simulink model "ball_balancing_omni3_multibody_lqi_rev1_r2024b"  (R2024b)
settings: Solver=VariableStepAuto  StartTime=0.0  StopTime=50  MaxStep=1e-3  MinStep=1e-6  RelTol=ballbotParams.simulation.relativeTolerance
PreLoadFcn:
  | if ~exist('ballbotParams','var'), ballbotParams = ballbotRev1Parameters; end
InitFcn:
  | if ~exist('ballbotParams','var') || ~isfield(ballbotParams,'parameterSource') || ballbotParams.parameterSource ~= "ballbotRev1Parameters" || ~isfield(ballbotParams,'controller') || ~isfield(ballbotParams,'estimator') || ~isfield(ballbotParams.controller,'torqueDrive') || ~isfield(ballbotParams.controller.torqueDrive,'propulsionGain') || ~isfield(ballbotParams.estimator,'truthDelaySteps') || ~isfield(ballbotParams.controller.torqueLqi,'robustness'), ballbotParams = ballbotRev1Parameters; end
  | % ballbotRev1RuntimeApply: re-apply runtime solver/driver/plant settings on every sim start.
  | clear functions;
  | ballbotRev1SimConfig;
  | if exist('ballbotParams','var'), ballbotRev1PlantAugment(bdroot, ballbotParams); end
values from neighbouring files (symbols this model uses):
  N = 0    [ballbotRollingResistance.m]
  s = result.spec    [ballbotBenchmark.m]
undefined symbols (not defined in the file or in its folder): ballbotCustomFriction, ballbotEstimatorInitialState, ballbotEstimatorUpdate, ballbotEulerToQuaternion, ballbotImuFromJoint, ballbotLqiControllerUpdate, ballbotLqiFeedbackState, ballbotMdd3aGateDrive, ballbotParams, ballbotPoseFromJoint, ballbotRev1CommandProfile, ballbotRollingResistance, ballbotRoverInitialPosition, ballbotShaftFrictionTorque, ballbotTorqueDutyStep, ballbotTruthGate, ballbotWheelRateFromDisplacement, X, Y, Z
libraries: nesl_utility x54, sm_lib x28, fl_lib x21, ee_lib x6
(part 1 of 3)
settings Model: Creator=cafdr  LastModifiedBy=cafdr
settings DataIOCC: LoggingIntervals=[-inf,inf]
settings ModelReferenceCC: UpdateModelReferenceTargets=IfOutOfDate
settings ConfigComp: CovBoundaryAbsTol=1.0e-5
settings SimscapeCC: SimscapeNominalValues="[{\"value\":\"1\",\"unit\":\"A\"},{\"value\":\"1\",\"unit\":\"bar\"},{\"value\":\"1\",\"unit\":\"cm^2\"},{\"value\":\"1\",\"unit\":\"cm^3/s\"},{\"value\":\"1\",\"unit\":\"kJ/kg\"},{\"value\":\"1\",\"unit\":\"kW\"},{\"value\":\"1\",\"unit\":\"l\"},{\"value\":\"1\",\"unit\":\"N\"},{\"value\":\"1\",\"unit\":\"N*m\"},{\"value\":\"1\",\"unit\":\"V\"},{\"value\":\"0.001\",\"unit\":\"Wb\"}]"  SimscapeLogDataHistory=10000
settings ExplorerConfigSet: InternalSimMechanicsExplorerSettings=|
  | <ExplorerConfiguration>
  | 
  |   <canonicalview>default</canonicalview>
  | 
  |   <TilePanel>
  |     <TileInfo>
  |       <Tiles Columns="1" Count="1" Height="986" Rows="1" Width="1142">
  |         <Row Weight="1"/>
  |         <Column Weight="1"/>
  |         <Tile Height="1" Width="1" X="0" Y="0"/>
  |       </Tiles>
  |     </TileInfo>
  |     <SceneInfo>
  |       <SceneViewer>
  |         <IsThisViewStd>
  |           <IsStandardView>off</IsStandardView>
  |           <StandardViewName>Front</StandardViewName>
  |         </IsThisViewStd>
  |         <BGColor>
  |           <R>1</R>
  |           <G>1</G>
  |           <B>1</B>
  |           <A>1</A>
  |         </BGColor>
  |         <Camera>
  |           <DoPerspective>off</DoPerspective>
  |           <Position>
  |             <X>1.5473752302641908</X>
  |             <Y>-7.8906176009490112</Y>
  |             <Z>3.2187132461389409</Z>
  |           </Position>
  |           <Center>
  |             <X>-0.24631476973580918</X>
  |             <Y>-0.11269760094901093</Y>
  |             <Z>0.28416324613894073</Z>
  |           </Center>
  |           <Up>
  |             <X>-0.21384970147003254</X>
  |             <Y>0.30128090391364881</Y>
  |             <Z>0.92924599655750617</Z>
  |           </Up>
  |           <XLim>0.70155682369920191</XLim>
  |           <YLim>0.70155682369920191</YLim>
  |           <ViewLimDist>0.01</ViewLimDist>
  |         </Camera>
  |       </SceneViewer>
  |     </SceneInfo>
  |   </TilePanel>
  | 
  |   <MechEditorPanel>
  |     <GfxPanelCameraMap/>
  |     <Cameras/>
  |     <VideoCreator>
  |       <IncludeTiles>All</IncludeTiles>
  |       <IncludeTime>on</IncludeTime>
  |       <IncludeWorldFrame>off</IncludeWorldFrame>
  |       <PlaybackSpeedRatio>1</PlaybackSpeedRatio>
  |       <FrameRate>30</FrameRate>
  |       <FrameSize>auto</FrameSize>
  |       <VideoFormat>UncompressedAVI</VideoFormat>
  |     </VideoCreator>
  |   </MechEditorPanel>
  | 
  |   <PlaybackSettings>
  |     <PlaybackSpeedFactor>1</PlaybackSpeedFactor>
  |   </PlaybackSettings>
  | 
  | </ExplorerConfiguration>

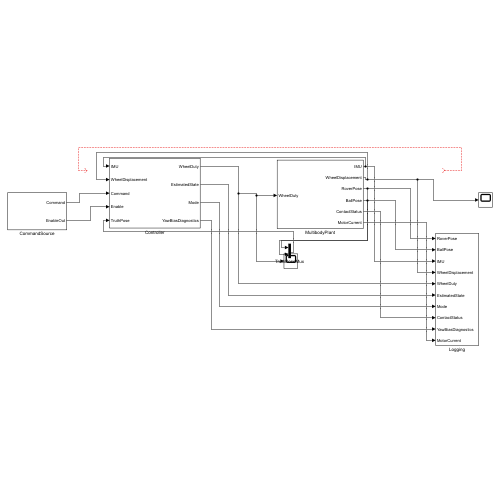
[thumbnail: Simulink's stored preview of the top-level diagram]
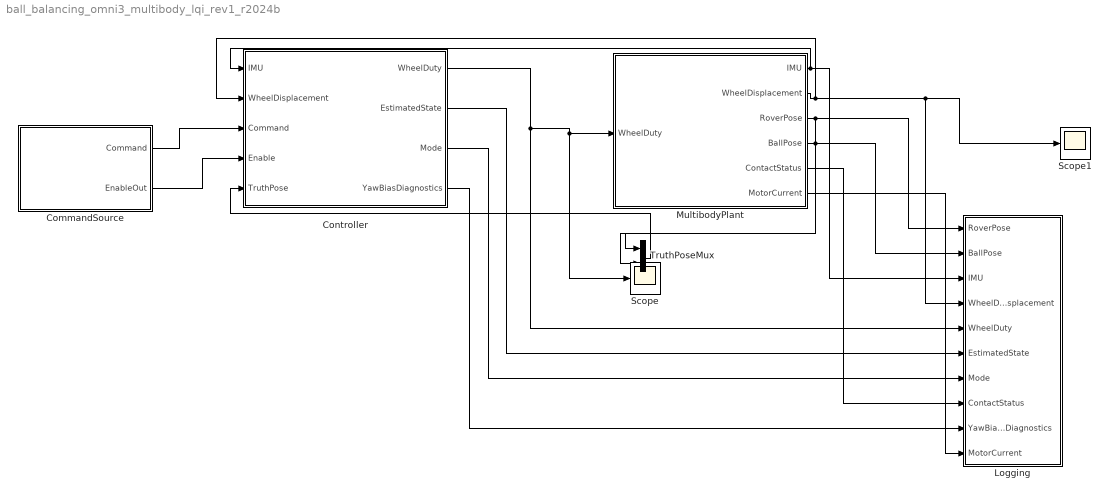
== system ball_balancing_omni3_multibody_lqi_rev1_r2024b ==
  CommandSource : Subsystem
  Controller : Subsystem
  Logging : Subsystem
  MultibodyPlant : Subsystem
  Scope : Scope
  Scope1 : Scope
  TruthPoseMux : Mux  Inputs=2
  wires:
  CommandSource/2(EnableOut) -> Controller/4(Enable)
  CommandSource/1(Command) -> Controller/3(Command)
  ? -> ?
  Controller/4(YawBiasDiagnostics) -> Logging/9(YawBiasDiagnostics)
  MultibodyPlant/2(WheelDisplacement) -> Logging/4(WheelDisplacement), Scope1/1, Controller/2(WheelDisplacement)
  MultibodyPlant/1(IMU) -> Logging/3(IMU), Controller/1(IMU)
  Controller/1(WheelDuty) -> Logging/5(WheelDuty), Scope/1, MultibodyPlant/1(WheelDuty)
  MultibodyPlant/3(RoverPose) -> Logging/1(RoverPose), TruthPoseMux/1
  MultibodyPlant/4(BallPose) -> Logging/2(BallPose), TruthPoseMux/2
  Controller/2(EstimatedState) -> Logging/6(EstimatedState)
  Controller/3(Mode) -> Logging/7(Mode)
  MultibodyPlant/5(ContactStatus) -> Logging/8(ContactStatus)
  MultibodyPlant/6(MotorCurrent) -> Logging/10(MotorCurrent)
  TruthPoseMux/1 -> Controller/5(TruthPose)

== system ball_balancing_omni3_multibody_lqi_rev1_r2024b/CommandSource ==
  CommandProfile : MATLABFcn  MATLABFcn=ballbotRev1CommandProfile(u,ballbotParams)  OutputDimensions=3
  Enable : Constant  Value=double(ballbotParams.command.enable)  SampleTime=ballbotParams.controller.sampleTime
  LogCommand : ToWorkspace  VariableName=velocityCommand  SaveFormat=Timeseries  SampleTime=-1
  SimulationTime : Clock
  Command : Outport
  EnableOut : Outport  Port=2
  wires:
  Enable/1 -> EnableOut/1
  SimulationTime/1 -> CommandProfile/1
  CommandProfile/1 -> LogCommand/1, Command/1

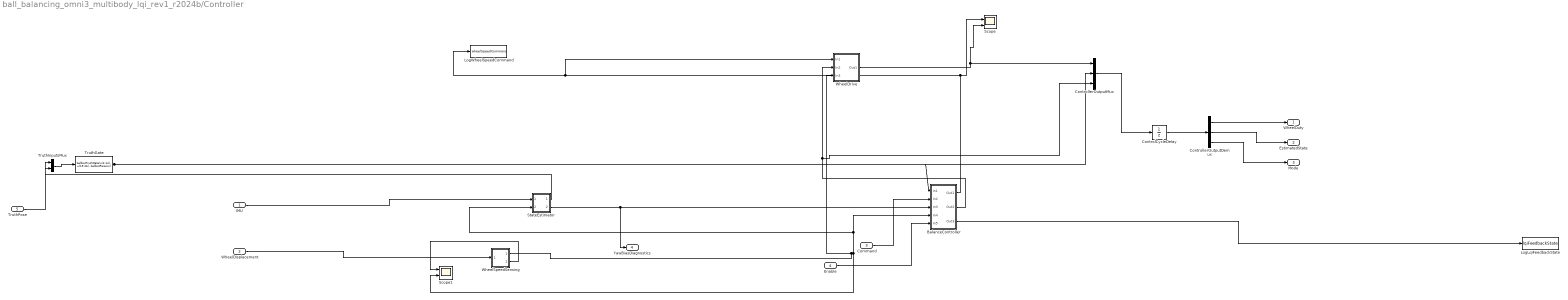
== system ball_balancing_omni3_multibody_lqi_rev1_r2024b/Controller ==
  IMU : Inport  PortDimensions=6
  WheelDisplacement : Inport  Port=2  PortDimensions=3
  Command : Inport  Port=3
  Enable : Inport  Port=4
  TruthPose : Inport  Port=5
  BalanceController : Subsystem
  ControlCycleDelay : UnitDelay  InitialCondition=zeros(18,1)  SampleTime=ballbotParams.controller.sampleTime
  ControllerOutputDemux : Demux  Outputs=[3 14 1]
  ControllerOutputMux : Mux  Inputs=3
  LogLqiFeedbackState : ToWorkspace  VariableName=lqiFeedbackState  SaveFormat=Timeseries  SampleTime=-1
  LogWheelSpeedCommand : ToWorkspace  VariableName=wheelSpeedCommand  SaveFormat=Timeseries  SampleTime=-1
  Scope : Scope  NumInputPorts=2
  Scope1 : Scope  NumInputPorts=2
  StateEstimator : Subsystem
  TruthGate : MATLABFcn  MATLABFcn=ballbotTruthGate(u(1:14), u(15:26), ballbotParams)  OutputDimensions=14  OutputSignalType=real  SampleTime=ballbotParams.controller.sampleTime
  TruthInputsMux : Mux  Inputs=2
  WheelDrive : Subsystem
  WheelSpeedSensing : Subsystem
  WheelDuty : Outport
  EstimatedState : Outport  Port=2
  Mode : Outport  Port=3
  YawBiasDiagnostics : Outport  Port=4
  wires:
  ControlCycleDelay/1 -> ControllerOutputDemux/1
  ControllerOutputDemux/3 -> Mode/1
  ControllerOutputDemux/1 -> WheelDuty/1
  ControllerOutputDemux/2 -> EstimatedState/1
  ControllerOutputMux/1 -> ControlCycleDelay/1
  WheelSpeedSensing/1(Out1) -> WheelDrive/3(In3), BalanceController/4(In4), StateEstimator/2(In2), Scope1/2
  WheelDisplacement/1 -> WheelSpeedSensing/1(In1)
  WheelSpeedSensing/2(Out2) -> Scope1/1
  StateEstimator/2(Out2) -> YawBiasDiagnostics/1, BalanceController/3(In3)
  IMU/1 -> StateEstimator/1(In1)
  BalanceController/1(Out1) -> WheelDrive/1(In1), LogWheelSpeedCommand/1, Scope/1
  BalanceController/2(Out2) -> WheelDrive/2(In2), ControllerOutputMux/3
  Command/1 -> BalanceController/2(In2)
  Enable/1 -> BalanceController/5(In5)
  BalanceController/3(Out3) -> LogLqiFeedbackState/1
  WheelDrive/1(Out1) -> Scope/2, ControllerOutputMux/1
  StateEstimator/1(Out1) -> TruthInputsMux/1
  TruthPose/1 -> TruthInputsMux/2
  TruthInputsMux/1 -> TruthGate/1
  TruthGate/1 -> BalanceController/1(In1), ControllerOutputMux/2

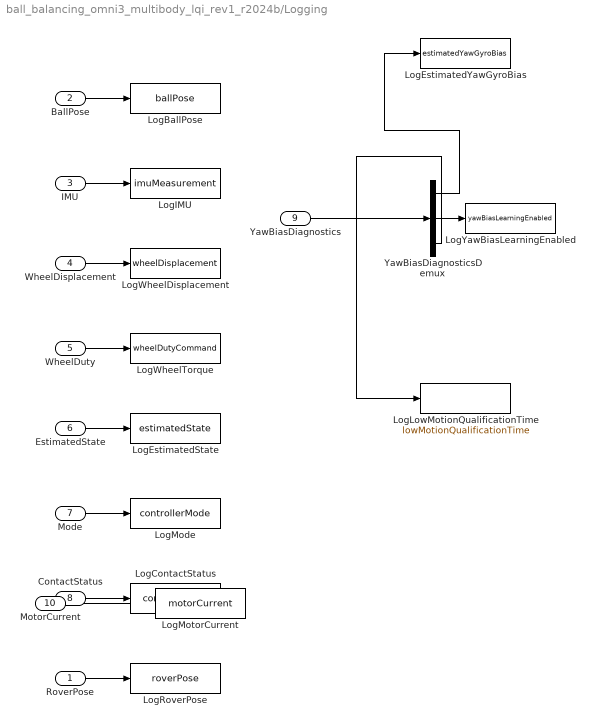
== system ball_balancing_omni3_multibody_lqi_rev1_r2024b/Logging ==
  RoverPose : Inport
  BallPose : Inport  Port=2
  IMU : Inport  Port=3
  WheelDisplacement : Inport  Port=4
  WheelDuty : Inport  Port=5
  EstimatedState : Inport  Port=6
  Mode : Inport  Port=7
  ContactStatus : Inport  Port=8
  YawBiasDiagnostics : Inport  Port=9
  MotorCurrent : Inport  Port=10
  LogBallPose : ToWorkspace  VariableName=ballPose  SaveFormat=Timeseries  SampleTime=-1
  LogContactStatus : ToWorkspace  VariableName=contactStatus  SaveFormat=Timeseries  SampleTime=-1
  LogEstimatedState : ToWorkspace  VariableName=estimatedState  SaveFormat=Timeseries  SampleTime=-1
  LogEstimatedYawGyroBias : ToWorkspace  VariableName=estimatedYawGyroBias  SaveFormat=Timeseries  SampleTime=-1
  LogIMU : ToWorkspace  VariableName=imuMeasurement  SaveFormat=Timeseries  SampleTime=-1
  LogLowMotionQualificationTime : ToWorkspace  VariableName=lowMotionQualificationTime  SaveFormat=Timeseries  SampleTime=-1
  LogMode : ToWorkspace  VariableName=controllerMode  SaveFormat=Timeseries  SampleTime=-1
  LogMotorCurrent : ToWorkspace  VariableName=motorCurrent  SaveFormat=Timeseries  SampleTime=-1
  LogRoverPose : ToWorkspace  VariableName=roverPose  SaveFormat=Timeseries  SampleTime=-1
  LogWheelDisplacement : ToWorkspace  VariableName=wheelDisplacement  SaveFormat=Timeseries  SampleTime=-1
  LogWheelTorque : ToWorkspace  VariableName=wheelDutyCommand  SaveFormat=Timeseries  SampleTime=-1
  LogYawBiasLearningEnabled : ToWorkspace  VariableName=yawBiasLearningEnabled  SaveFormat=Timeseries  SampleTime=-1
  YawBiasDiagnosticsDemux : Demux  Outputs=3
  wires:
  ContactStatus/1 -> LogContactStatus/1
  Mode/1 -> LogMode/1
  EstimatedState/1 -> LogEstimatedState/1
  WheelDuty/1 -> LogWheelTorque/1
  WheelDisplacement/1 -> LogWheelDisplacement/1
  IMU/1 -> LogIMU/1
  BallPose/1 -> LogBallPose/1
  RoverPose/1 -> LogRoverPose/1
  YawBiasDiagnosticsDemux/3 -> LogLowMotionQualificationTime/1
  YawBiasDiagnosticsDemux/2 -> LogYawBiasLearningEnabled/1
  YawBiasDiagnosticsDemux/1 -> LogEstimatedYawGyroBias/1
  YawBiasDiagnostics/1 -> YawBiasDiagnosticsDemux/1
  MotorCurrent/1 -> LogMotorCurrent/1

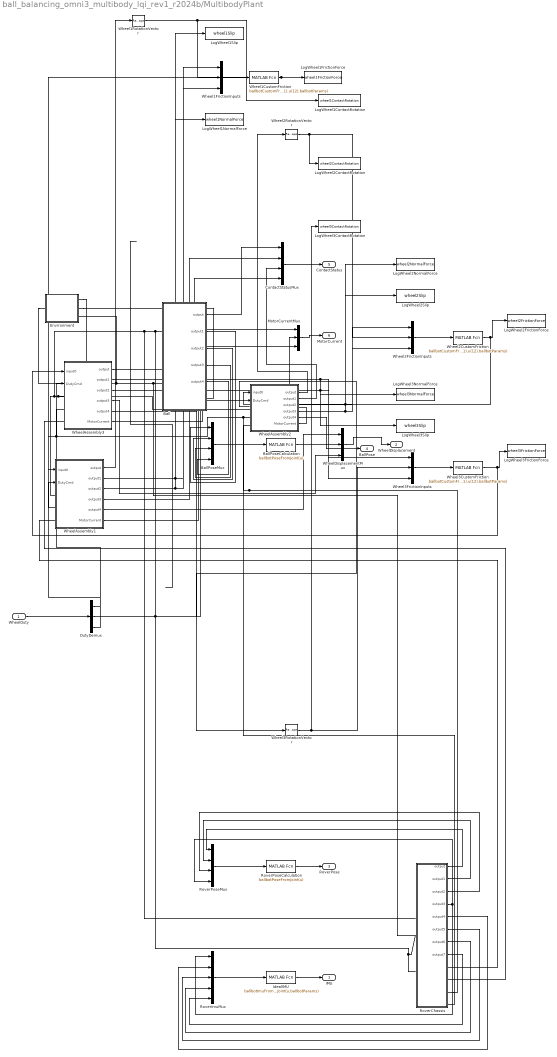
== system ball_balancing_omni3_multibody_lqi_rev1_r2024b/MultibodyPlant ==
  WheelDuty : Inport
  Ball : Subsystem
  BallPoseCalculation : MATLABFcn  MATLABFcn=ballbotPoseFromJoint(u)  OutputDimensions=6
  BallPoseMux : Mux
  ContactStatusMux : Mux
  DutyDemux : Demux  Outputs=3
  Environment : Subsystem
  IdealIMU : MATLABFcn  MATLABFcn=ballbotImuFromJoint(u,ballbotParams)  OutputDimensions=6  SampleTime=ballbotParams.estimator.sampleTime
  LogWheel1ContactRotation : ToWorkspace  VariableName=wheel1ContactRotation  SaveFormat=Timeseries  SampleTime=-1
  LogWheel1FrictionForce : ToWorkspace  VariableName=wheel1FrictionForce  SaveFormat=Timeseries  SampleTime=-1
  LogWheel1NormalForce : ToWorkspace  VariableName=wheel1NormalForce  SaveFormat=Timeseries  SampleTime=-1
  LogWheel1Slip : ToWorkspace  VariableName=wheel1Slip  SaveFormat=Timeseries  SampleTime=-1
  LogWheel2ContactRotation : ToWorkspace  VariableName=wheel2ContactRotation  SaveFormat=Timeseries  SampleTime=-1
  LogWheel2FrictionForce : ToWorkspace  VariableName=wheel2FrictionForce  SaveFormat=Timeseries  SampleTime=-1
  LogWheel2NormalForce : ToWorkspace  VariableName=wheel2NormalForce  SaveFormat=Timeseries  SampleTime=-1
  LogWheel2Slip : ToWorkspace  VariableName=wheel2Slip  SaveFormat=Timeseries  SampleTime=-1
  LogWheel3ContactRotation : ToWorkspace  VariableName=wheel3ContactRotation  SaveFormat=Timeseries  SampleTime=-1
  LogWheel3FrictionForce : ToWorkspace  VariableName=wheel3FrictionForce  SaveFormat=Timeseries  SampleTime=-1
  LogWheel3NormalForce : ToWorkspace  VariableName=wheel3NormalForce  SaveFormat=Timeseries  SampleTime=-1
  LogWheel3Slip : ToWorkspace  VariableName=wheel3Slip  SaveFormat=Timeseries  SampleTime=-1
  MotorCurrentMux : Mux  Inputs=3
  RoverChassis : Subsystem
  RoverImuMux : Mux  Inputs=5
  RoverPoseCalculation : MATLABFcn  MATLABFcn=ballbotPoseFromJoint(u)  OutputDimensions=6
  RoverPoseMux : Mux
  Wheel1CustomFriction : MATLABFcn  MATLABFcn=ballbotCustomFriction(u(1:2),u(3:11),u(12),ballbotParams)  OutputDimensions=2
  Wheel1FrictionInputs : Mux  Inputs=3
  Wheel1RotationVector : Reshape
  Wheel2CustomFriction : MATLABFcn  MATLABFcn=ballbotCustomFriction(u(1:2),u(3:11),u(12),ballbotParams)  OutputDimensions=2
  Wheel2FrictionInputs : Mux  Inputs=3
  Wheel2RotationVector : Reshape
  Wheel3CustomFriction : MATLABFcn  MATLABFcn=ballbotCustomFriction(u(1:2),u(3:11),u(12),ballbotParams)  OutputDimensions=2
  Wheel3FrictionInputs : Mux  Inputs=3
  Wheel3RotationVector : Reshape
  WheelAssembly1 : Subsystem
  WheelAssembly2 : Subsystem
  WheelAssembly3 : Subsystem
  WheelDisplacementMux : Mux  Inputs=3
  IMU : Outport
  WheelDisplacement : Outport  Port=2
  RoverPose : Outport  Port=3
  BallPose : Outport  Port=4
  ContactStatus : Outport  Port=5
  MotorCurrent : Outport  Port=6
  wires:
  ContactStatusMux/1 -> ContactStatus/1
  BallPoseMux/1 -> BallPoseCalculation/1
  RoverPoseCalculation/1 -> RoverPose/1
  RoverPoseMux/1 -> RoverPoseCalculation/1
  IdealIMU/1 -> IMU/1
  RoverImuMux/1 -> IdealIMU/1
  DutyDemux/2 -> WheelAssembly2/2(DutyCmd)
  WheelDuty/1 -> DutyDemux/1
  Wheel1FrictionInputs/1 -> Wheel1CustomFriction/1
  Wheel3FrictionInputs/1 -> Wheel3CustomFriction/1
  Wheel2CustomFriction/1 -> WheelAssembly2/1(input0), LogWheel2FrictionForce/1
  Wheel2FrictionInputs/1 -> Wheel2CustomFriction/1
  Wheel1RotationVector/1 -> Wheel1FrictionInputs/2, LogWheel1ContactRotation/1
  Wheel2RotationVector/1 -> Wheel2FrictionInputs/2, LogWheel2ContactRotation/1
  Wheel3RotationVector/1 -> Wheel3FrictionInputs/2, LogWheel3ContactRotation/1
  Ball/1(output) -> ContactStatusMux/1
  Ball/2(output1) -> BallPoseMux/1
  Ball/3(output2) -> BallPoseMux/2
  Ball/4(output3) -> BallPoseMux/3
  Ball/5(output4) -> BallPoseMux/4
  WheelAssembly2/3(output2) -> LogWheel2NormalForce/1, Wheel2FrictionInputs/3
  WheelAssembly2/4(output3) -> LogWheel2Slip/1, Wheel2FrictionInputs/1
  WheelAssembly2/1(output) -> Wheel2RotationVector/1
  WheelAssembly2/2(output1) -> ContactStatusMux/3
  WheelAssembly2/6(MotorCurrent) -> MotorCurrentMux/2
  MotorCurrentMux/1 -> MotorCurrent/1
  RoverChassis/8(output7) -> RoverImuMux/5
  RoverChassis/7(output6) -> RoverImuMux/4
  RoverChassis/6(output5) -> RoverImuMux/3
  RoverChassis/5(output4) -> RoverImuMux/2
  RoverChassis/3(output2) -> RoverPoseMux/3
  RoverChassis/2(output1) -> RoverPoseMux/2
  RoverChassis/1(output) -> RoverPoseMux/1
  RoverChassis/4(output3) -> RoverPoseMux/4, RoverImuMux/1
  WheelAssembly3/6(MotorCurrent) -> MotorCurrentMux/3
  WheelAssembly1/6(MotorCurrent) -> MotorCurrentMux/1
  WheelAssembly3/5(output4) -> Wheel3RotationVector/1
  WheelAssembly3/1(output) -> ContactStatusMux/4
  WheelAssembly3/3(output2) -> Wheel3FrictionInputs/1, LogWheel3Slip/1
  WheelAssembly3/2(output1) -> Wheel3FrictionInputs/3, LogWheel3NormalForce/1
  WheelAssembly1/4(output3) -> ContactStatusMux/2
  WheelAssembly1/1(output) -> Wheel1RotationVector/1
  WheelAssembly1/3(output2) -> LogWheel1Slip/1, Wheel1FrictionInputs/1
  WheelAssembly1/2(output1) -> Wheel1FrictionInputs/3, LogWheel1NormalForce/1
  Wheel3CustomFriction/1 -> WheelAssembly3/1(input0), LogWheel3FrictionForce/1
  Wheel1CustomFriction/1 -> LogWheel1FrictionForce/1, WheelAssembly1/1(input0)
  DutyDemux/1 -> WheelAssembly1/2(DutyCmd)
  DutyDemux/3 -> WheelAssembly3/2(DutyCmd)
  BallPoseCalculation/1 -> BallPose/1
  WheelDisplacementMux/1 -> WheelDisplacement/1
  WheelAssembly2/5(output4) -> WheelDisplacementMux/2
  WheelAssembly3/4(output3) -> WheelDisplacementMux/3
  WheelAssembly1/5(output4) -> WheelDisplacementMux/1
  connections:
  Environment/RConn2 -- Ball/RConn1
  Environment/LConn1 -- Ball/LConn2 -- RoverChassis/LConn1 -- Environment/RConn3 -- Environment/RConn1
  ?
  ?
  WheelAssembly2/LConn3 -- RoverChassis/RConn4
  WheelAssembly2/LConn1 -- WheelAssembly1/LConn1 -- Ball/LConn1 -- WheelAssembly3/LConn1
  RoverChassis/RConn3 -- WheelAssembly3/LConn2 -- WheelAssembly1/LConn2 -- WheelAssembly2/LConn2
  WheelAssembly1/LConn3 -- RoverChassis/RConn1
  WheelAssembly3/LConn3 -- RoverChassis/RConn2

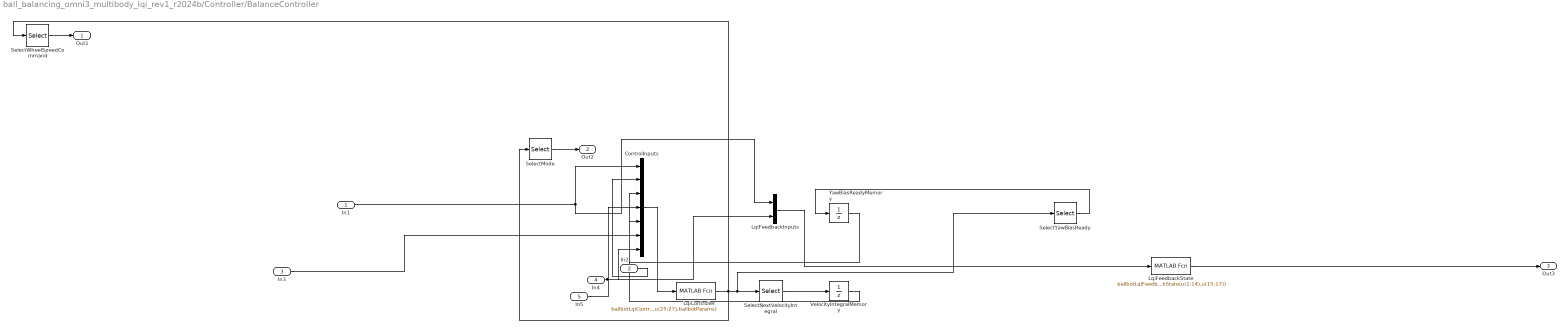
== system ball_balancing_omni3_multibody_lqi_rev1_r2024b/Controller/BalanceController ==
  In1 : Inport
  In2 : Inport  Port=2
  In3 : Inport  Port=3
  In4 : Inport  Port=4
  In5 : Inport  Port=5
  ControlInputs : Mux  Inputs=7
  LqiController : MATLABFcn  MATLABFcn=ballbotLqiControllerUpdate(u(1:14),u(15:17),u(18:19),u(20),u(21),u(22:24),u(25:27),ballbotParams)  OutputDimensions=7  SampleTime=ballbotParams.controller.sampleTime
  LqiFeedbackInputs : Mux  Inputs=2
  LqiFeedbackState : MATLABFcn  MATLABFcn=ballbotLqiFeedbackState(u(1:14),u(15:17))  OutputDimensions=10
  SelectMode : Selector  InputPortWidth=7  IndexOptions=Index vector (dialog)  Indices=6  OutputSizes=1
  SelectNextVelocityIntegral : Selector  InputPortWidth=7  IndexOptions=Index vector (dialog)  Indices=4:5  OutputSizes=1
  SelectWheelSpeedCommand : Selector  InputPortWidth=7  IndexOptions=Index vector (dialog)  Indices=1:3  OutputSizes=1
  SelectYawBiasReady : Selector  InputPortWidth=7  IndexOptions=Index vector (dialog)  Indices=7  OutputSizes=1
  VelocityIntegralMemory : UnitDelay  InitialCondition=zeros(2,1)  SampleTime=ballbotParams.controller.sampleTime
  YawBiasReadyMemory : UnitDelay  SampleTime=ballbotParams.controller.sampleTime
  Out1 : Outport
  Out2 : Outport  Port=2
  Out3 : Outport  Port=3
  wires:
  SelectNextVelocityIntegral/1 -> VelocityIntegralMemory/1
  LqiController/1 -> SelectYawBiasReady/1, SelectNextVelocityIntegral/1, SelectWheelSpeedCommand/1, SelectMode/1
  LqiFeedbackInputs/1 -> LqiFeedbackState/1
  In1/1 -> LqiFeedbackInputs/1, ControlInputs/1
  VelocityIntegralMemory/1 -> ControlInputs/3
  SelectYawBiasReady/1 -> YawBiasReadyMemory/1
  YawBiasReadyMemory/1 -> ControlInputs/5
  SelectWheelSpeedCommand/1 -> Out1/1
  In3/1 -> ControlInputs/6
  ControlInputs/1 -> LqiController/1
  In5/1 -> ControlInputs/4
  In4/1 -> LqiFeedbackInputs/2, ControlInputs/7
  LqiFeedbackState/1 -> Out3/1
  SelectMode/1 -> Out2/1
  In2/1 -> ControlInputs/2

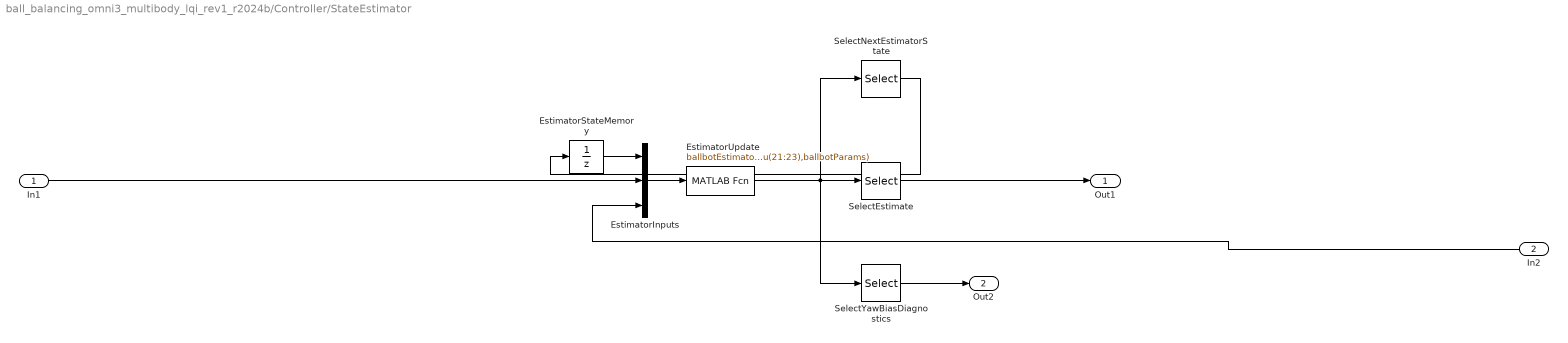
== system ball_balancing_omni3_multibody_lqi_rev1_r2024b/Controller/StateEstimator ==
  In1 : Inport
  In2 : Inport  Port=2
  EstimatorInputs : Mux  Inputs=3
  EstimatorStateMemory : UnitDelay  InitialCondition=ballbotEstimatorInitialState(ballbotParams)  SampleTime=ballbotParams.controller.sampleTime
  EstimatorUpdate : MATLABFcn  MATLABFcn=ballbotEstimatorUpdate(u(1:14),u(15:20),u(21:23),ballbotParams)  OutputDimensions=31  SampleTime=ballbotParams.controller.sampleTime
  SelectEstimate : Selector  InputPortWidth=31  IndexOptions=Index vector (dialog)  Indices=15:28  OutputSizes=1
  SelectNextEstimatorState : Selector  InputPortWidth=31  IndexOptions=Index vector (dialog)  Indices=1:14  OutputSizes=1
  SelectYawBiasDiagnostics : Selector  InputPortWidth=31  IndexOptions=Index vector (dialog)  Indices=29:31  OutputSizes=1
  Out1 : Outport
  Out2 : Outport  Port=2
  wires:
  SelectYawBiasDiagnostics/1 -> Out2/1
  EstimatorUpdate/1 -> SelectEstimate/1, SelectNextEstimatorState/1, SelectYawBiasDiagnostics/1
  In2/1 -> EstimatorInputs/3
  SelectNextEstimatorState/1 -> EstimatorStateMemory/1
  EstimatorStateMemory/1 -> EstimatorInputs/1
  SelectEstimate/1 -> Out1/1
  EstimatorInputs/1 -> EstimatorUpdate/1
  In1/1 -> EstimatorInputs/2

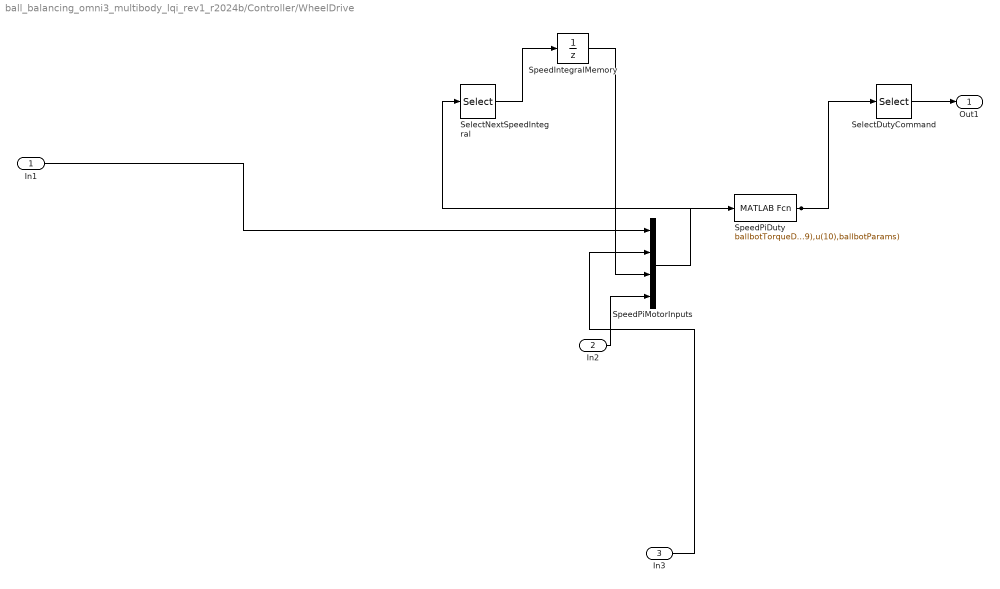
== system ball_balancing_omni3_multibody_lqi_rev1_r2024b/Controller/WheelDrive ==
  In1 : Inport
  In2 : Inport  Port=2
  In3 : Inport  Port=3
  SelectDutyCommand : Selector  InputPortWidth=6  IndexOptions=Index vector (dialog)  Indices=1:3  OutputSizes=1
  SelectNextSpeedIntegral : Selector  InputPortWidth=6  IndexOptions=Index vector (dialog)  Indices=4:6  OutputSizes=1
  SpeedIntegralMemory : UnitDelay  InitialCondition=zeros(3,1)  SampleTime=ballbotParams.controller.sampleTime
  SpeedPiDuty : MATLABFcn  MATLABFcn=ballbotTorqueDutyStep(u(1:3),u(4:6),u(7:9),u(10),ballbotParams)  OutputDimensions=6  SampleTime=ballbotParams.controller.sampleTime
  SpeedPiMotorInputs : Mux
  Out1 : Outport
  wires:
  SelectNextSpeedIntegral/1 -> SpeedIntegralMemory/1
  SpeedPiMotorInputs/1 -> SpeedPiDuty/1
  SpeedPiDuty/1 -> SelectDutyCommand/1, SelectNextSpeedIntegral/1
  SelectDutyCommand/1 -> Out1/1
  In2/1 -> SpeedPiMotorInputs/4
  In1/1 -> SpeedPiMotorInputs/1
  SpeedIntegralMemory/1 -> SpeedPiMotorInputs/3
  In3/1 -> SpeedPiMotorInputs/2

== system ball_balancing_omni3_multibody_lqi_rev1_r2024b/Controller/WheelSpeedSensing ==
  In1 : Inport
  PreviousWheelDisplacement : UnitDelay  InitialCondition=zeros(3,1)  SampleTime=ballbotParams.controller.sampleTime
  WheelRateCalculation : MATLABFcn  MATLABFcn=ballbotWheelRateFromDisplacement(u(1:3),u(4:6),ballbotParams.estimator.sampleTime,ballbotParams.encoder.quantization)  OutputDimensions=3  SampleTime=ballbotParams.controller.sampleTime
  WheelRateInputs : Mux  Inputs=2
  Out1 : Outport
  Out2 : Outport  Port=2
  wires:
  In1/1 -> WheelRateInputs/1, PreviousWheelDisplacement/1
  WheelRateCalculation/1 -> Out1/1
  WheelRateInputs/1 -> WheelRateCalculation/1
  PreviousWheelDisplacement/1 -> Out2/1, WheelRateInputs/2

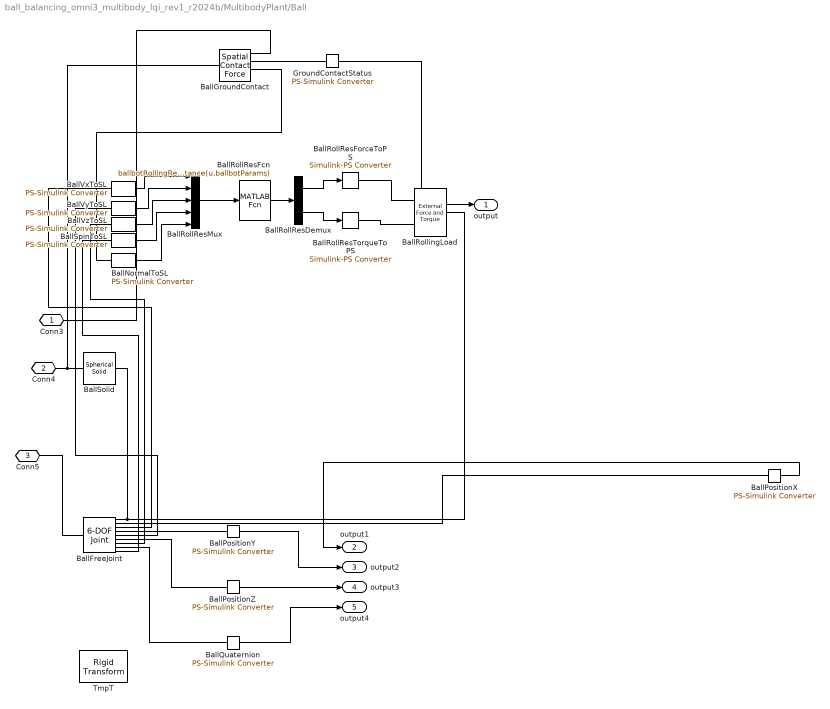
== system ball_balancing_omni3_multibody_lqi_rev1_r2024b/MultibodyPlant/Ball ==
  BallFreeJoint : sm_lib/Joints/6-DOF Joint  JointMode=Normal  CompositeWrenchDir=FollowerOnBase  CompositeWrenchFrame=BaseFrame  SenseConstraintForce=off  SenseConstraintTorque=off  SenseTotalForce=off  SenseTotalTorque=off  PxPositionTargetSpecify=on  PxPositionTargetPriority=High  PxPositionTargetValue=ballbotParams.rover.initialPositionWorld(1)  PxPositionTargetValueUnits=m  PxVelocityTargetSpecify=off  PxVelocityTargetPriority=High  PxVelocityTargetValue=0  PxVelocityTargetValueUnits=m/s  PxEquilibriumPosition=0  PxEquilibriumPositionUnits=m  PxSpringStiffness=0  PxSpringStiffnessUnits=N/m  PxDampingCoefficient=0  PxDampingCoefficientUnits=N/(m/s)  PxLowerLimitSpecify=off  PxLowerLimitBound=-1  PxLowerLimitBoundUnits=m  PxLowerLimitStiffness=1e6  PxLowerLimitStiffnessUnits=N/m  PxLowerLimitDamping=1e3  PxLowerLimitDampingUnits=N/(m/s)  PxLowerLimitTransitionRegionWidth=1e-4  PxLowerLimitTransitionRegionWidthUnits=m  PxUpperLimitSpecify=off  PxUpperLimitBound=1  PxUpperLimitBoundUnits=m  PxUpperLimitStiffness=1e6  PxUpperLimitStiffnessUnits=N/m  PxUpperLimitDamping=1e3  PxUpperLimitDampingUnits=N/(m/s)  PxUpperLimitTransitionRegionWidth=1e-4  PxUpperLimitTransitionRegionWidthUnits=m  PxTorqueActuationMode=NoTorque  PxMotionActuationMode=ComputedMotion  PxSensePosition=on  PxSenseVelocity=on  PxSenseAcceleration=off  PxSenseTorqueForce=off  PxSenseLowerLimitTorqueForce=off  PxSenseUpperLimitTorqueForce=off  PyPositionTargetSpecify=on  PyPositionTargetPriority=High  PyPositionTargetValue=ballbotParams.rover.initialPositionWorld(2)  PyPositionTargetValueUnits=m  PyVelocityTargetSpecify=off  PyVelocityTargetPriority=High  PyVelocityTargetValue=0  PyVelocityTargetValueUnits=m/s  PyEquilibriumPosition=0  PyEquilibriumPositionUnits=m  PySpringStiffness=0  PySpringStiffnessUnits=N/m  PyDampingCoefficient=0  PyDampingCoefficientUnits=N/(m/s)  PyLowerLimitSpecify=off  PyLowerLimitBound=-1  PyLowerLimitBoundUnits=m  PyLowerLimitStiffness=1e6  PyLowerLimitStiffnessUnits=N/m  PyLowerLimitDamping=1e3  PyLowerLimitDampingUnits=N/(m/s)  PyLowerLimitTransitionRegionWidth=1e-4  PyLowerLimitTransitionRegionWidthUnits=m  PyUpperLimitSpecify=off  PyUpperLimitBound=1  PyUpperLimitBoundUnits=m  PyUpperLimitStiffness=1e6  PyUpperLimitStiffnessUnits=N/m  PyUpperLimitDamping=1e3  PyUpperLimitDampingUnits=N/(m/s)  PyUpperLimitTransitionRegionWidth=1e-4  PyUpperLimitTransitionRegionWidthUnits=m  PyTorqueActuationMode=NoTorque  PyMotionActuationMode=ComputedMotion  PySensePosition=on  PySenseVelocity=on  PySenseAcceleration=off  PySenseTorqueForce=off  PySenseLowerLimitTorqueForce=off  PySenseUpperLimitTorqueForce=off  PzPositionTargetSpecify=on  PzPositionTargetPriority=High  PzPositionTargetValue=ballbotParams.rover.initialPositionWorld(3)-ballbotParams.rover.centerAboveBall  PzPositionTargetValueUnits=m  PzVelocityTargetSpecify=off  PzVelocityTargetPriority=High  PzVelocityTargetValue=0  PzVelocityTargetValueUnits=m/s  PzEquilibriumPosition=0  PzEquilibriumPositionUnits=m  PzSpringStiffness=0  PzSpringStiffnessUnits=N/m  PzDampingCoefficient=0  PzDampingCoefficientUnits=N/(m/s)  PzLowerLimitSpecify=off  PzLowerLimitBound=-1  PzLowerLimitBoundUnits=m  PzLowerLimitStiffness=1e6  PzLowerLimitStiffnessUnits=N/m  PzLowerLimitDamping=1e3  PzLowerLimitDampingUnits=N/(m/s)  PzLowerLimitTransitionRegionWidth=1e-4  PzLowerLimitTransitionRegionWidthUnits=m  PzUpperLimitSpecify=off  PzUpperLimitBound=1  PzUpperLimitBoundUnits=m  PzUpperLimitStiffness=1e6  PzUpperLimitStiffnessUnits=N/m  PzUpperLimitDamping=1e3  PzUpperLimitDampingUnits=N/(m/s)  PzUpperLimitTransitionRegionWidth=1e-4  PzUpperLimitTransitionRegionWidthUnits=m  PzTorqueActuationMode=NoTorque  PzMotionActuationMode=ComputedMotion  PzSensePosition=on  PzSenseVelocity=on  PzSenseAcceleration=off  PzSenseTorqueForce=off  PzSenseLowerLimitTorqueForce=off  PzSenseUpperLimitTorqueForce=off  SphPositionTargetSpecify=on  SphPositionTargetPriority=High  SphPositionTargetRotationMethod=Quaternion  SphPositionTargetFollAlignAxisA=+X  SphPositionTargetBaseAlignAxisA=+Y  SphPositionTargetFollAlignAxisB=+Y  SphPositionTargetBaseAlignAxisB=+Z  SphPositionTargetRotationStandardAxis=+Z  SphPositionTargetRotationAngle=0  SphPositionTargetRotationAngleUnits=deg  SphPositionTargetRotationArbitraryAxis=[0 0 1]  SphPositionTargetRotationSequenceAxes=FollowerAxes  SphPositionTargetRotationSequence=XYX  SphPositionTargetRotationSequenceAngles=[0 0 0]  SphPositionTargetRotationSequenceAnglesUnits=deg  SphPositionTargetRotationMatrix=[1 0 0;0 1 0;0 0 1]  SphPositionTargetQuaternion=[1 0 0 0]  SphVelocityTargetSpecify=off  SphVelocityTargetPriority=High  SphVelocityTargetValue=[0 0 0]  SphVelocityTargetValueUnits=deg/s  SphVelocityTargetInFollowerFrame=on  SphEqPosRotationMethod=None  SphEqPosFollAlignAxisA=+X  SphEqPosBaseAlignAxisA=+Y  SphEqPosFollAlignAxisB=+Y  SphEqPosBaseAlignAxisB=+Z  SphEqPosRotationStandardAxis=+Z  SphEqPosRotationAngle=0  SphEqPosRotationAngleUnits=deg  SphEqPosRotationArbitraryAxis=[0 0 1]  SphEqPosRotationSequenceAxes=FollowerAxes  SphEqPosRotationSequence=XYX  SphEqPosRotationSequenceAngles=[0 0 0]  SphEqPosRotationSequenceAnglesUnits=deg  SphEqPosRotationMatrix=[1 0 0;0 1 0;0 0 1]  SphEqPosQuaternion=[1 0 0 0]  SphSpringStiffness=0  SphSpringStiffnessUnits=N*m/deg  SphDampingCoefficient=0  SphDampingCoefficientUnits=N*m/(deg/s)  SphLowerLimitSpecify=off  SphLowerLimitBound=15  SphLowerLimitBoundUnits=deg  SphLowerLimitStiffness=1e4  SphLowerLimitStiffnessUnits=N*m/deg  SphLowerLimitDamping=10  SphLowerLimitDampingUnits=N*m/(deg/s)  SphLowerLimitTransitionRegionWidth=0.1  SphLowerLimitTransitionRegionWidthUnits=deg  SphUpperLimitSpecify=off  SphUpperLimitBound=45  SphUpperLimitBoundUnits=deg  SphUpperLimitStiffness=1e4  SphUpperLimitStiffnessUnits=N*m/deg  SphUpperLimitDamping=10  SphUpperLimitDampingUnits=N*m/(deg/s)  SphUpperLimitTransitionRegionWidth=0.1  SphUpperLimitTransitionRegionWidthUnits=deg  SphTorqueActuationMode=NoTorque  SphActuateTorqueX=off  SphActuateTorqueY=off  SphActuateTorqueZ=off  SphActuateTorque=off  SphActuationFrame=BaseFrame  SphSensePosition=on  SphSenseVelocityX=off  SphSenseVelocityY=off  SphSenseVelocityZ=off  SphSenseVelocity=on  SphSenseAccelerationX=off  SphSenseAccelerationY=off  SphSenseAccelerationZ=off  SphSenseAcceleration=off  SphSenseLowerLimitTorqueMag=off  SphSenseUpperLimitTorqueMag=off  SphSensingFrame=BaseFrame
  BallGroundContact : sm_lib/Forces and Torques/Spatial Contact Force  SenseSeparationDistance=off  NormalForceType=SmoothSpringDamper  NormalStiffness=ballbotParams.contact.ballGround.normalStiffness  NormalStiffnessUnits=N/m  NormalDamping=ballbotParams.contact.ballGround.normalDamping  NormalDampingUnits=N/(m/s)  NormalTransitionRegionWidth=ballbotParams.contact.ballGround.transitionWidth  NormalTransitionRegionWidthUnits=m  FrictionType=SmoothStickSlip  CoefficientOfStaticFriction=ballbotParams.contact.ballGround.staticFriction  CoefficientOfDynamicFriction=ballbotParams.contact.ballGround.dynamicFriction  FrictionalCriticalVelocity=ballbotParams.contact.ballGround.criticalVelocity  FrictionalCriticalVelocityUnits=m/s  SenseContactSignal=on  SensePenetrationDepth=off  SenseNormalVelocity=off  SenseTangentialVelocity=on  SensingForceTorqueDirection=BaseOnFollower  SensingForceTorqueResolutionFrame=ContactFrame  SenseNormalForce=off  SenseNormalForceMagnitude=on  SenseNormalTorque=off  SenseFrictionalForce=off  SenseFrictionalForceMagnitude=off  SenseFrictionalTorque=off  SenseTotalForce=off  SenseTotalTorque=off  SenseContactBaseRotation=off  SenseContactBaseTranslation=off  SenseContactFollowerRotation=off  SenseContactFollowerTranslation=off  ZeroCrossDetectContactStartAndEnd=on
  BallNormalToSL : nesl_utility/PS-Simulink Converter  PhysicalDomain=network_engine_domain  SubClassName=ps_output  LeftPortType=input  RightPortType=output  PseudoPeriodic=off  Frequencies=[]  VectorFormat=inherit  Unit=N  AffineConversion=off
  BallPositionX : nesl_utility/PS-Simulink Converter  PhysicalDomain=network_engine_domain  SubClassName=ps_output  LeftPortType=input  RightPortType=output  PseudoPeriodic=off  Frequencies=[]  VectorFormat=inherit  Unit=m  AffineConversion=off
  BallPositionY : nesl_utility/PS-Simulink Converter  PhysicalDomain=network_engine_domain  SubClassName=ps_output  LeftPortType=input  RightPortType=output  PseudoPeriodic=off  Frequencies=[]  VectorFormat=inherit  Unit=m  AffineConversion=off
  BallPositionZ : nesl_utility/PS-Simulink Converter  PhysicalDomain=network_engine_domain  SubClassName=ps_output  LeftPortType=input  RightPortType=output  PseudoPeriodic=off  Frequencies=[]  VectorFormat=inherit  Unit=m  AffineConversion=off
  BallQuaternion : nesl_utility/PS-Simulink Converter  PhysicalDomain=network_engine_domain  SubClassName=ps_output  LeftPortType=input  RightPortType=output  PseudoPeriodic=off  Frequencies=[]  VectorFormat=inherit  Unit=1  AffineConversion=off
  BallRollResDemux : Demux  Outputs=[3 3]
  BallRollResFcn : MATLABFcn  MATLABFcn=ballbotRollingResistance(u,ballbotParams)
  BallRollResForceToPS : nesl_utility/Simulink-PS Converter  PhysicalDomain=network_engine_domain  SubClassName=ps_input  LeftPortType=input  RightPortType=output  PseudoPeriodic=off  Frequencies=[]  NoiseDistribution=none  NoiseParameters=[]  Unit=N  AffineConversion=off  FilteringAndDerivatives=provide  SimscapeFilterOrder=1  InputFilterTimeConstant=0.001  UdotUserProvided=0
  BallRollResMux : Mux  Inputs=5
  BallRollResTorqueToPS : nesl_utility/Simulink-PS Converter  PhysicalDomain=network_engine_domain  SubClassName=ps_input  LeftPortType=input  RightPortType=output  PseudoPeriodic=off  Frequencies=[]  NoiseDistribution=none  NoiseParameters=[]  Unit=N*m  AffineConversion=off  FilteringAndDerivatives=provide  SimscapeFilterOrder=1  InputFilterTimeConstant=0.001  UdotUserProvided=0
  BallRollingLoad : sm_lib/Forces and Torques/External Force and Torque  EnableForceX=off  EnableForceY=off  EnableForceZ=off  EnableForce=on  ForceResolutionFrame=World  EnableTorqueX=off  EnableTorqueY=off  EnableTorqueZ=off  EnableTorque=on  TorqueResolutionFrame=World
  BallSolid : sm_lib/Body Elements/Spherical Solid  SphereRadius=ballbotParams.ball.radius  SphereRadiusUnits=m  ExportEntireGeometry=on  InertiaType=Custom  BasedOnType=Mass  Density=1000  DensityUnits=kg/m^3  Mass=ballbotParams.ball.mass  MassUnits=kg  CenterOfMass=[0 0 0]  CenterOfMassUnits=m  MomentsOfInertia=[ballbotParams.ball.inertia(1,1) ballbotParams.ball.inertia(2,2) ballbotParams.ball.inertia(3,3)]  MomentsOfInertiaUnits=kg*m^2  ProductsOfInertia=[0 0 0]  ProductsOfInertiaUnits=kg*m^2  GraphicType=FromGeometry  MarkerShape=Sphere  MarkerSize=10  GraphicVisPropType=SimpleVisualProperties  GraphicDiffuseColor=[0.15 0.35 0.85 1.0]  GraphicOpacity=1  GraphicSpecularColor=[0.5 0.5 0.5 1.0]  GraphicAmbientColor=[0.15 0.15 0.15 1.0]  GraphicEmissiveColor=[0.0 0.0 0.0 1.0]  GraphicShininess=75  DoExposeReferenceFrame=on  SerializedFrames=<Frames/>
  BallSpinToSL : nesl_utility/PS-Simulink Converter  PhysicalDomain=network_engine_domain  SubClassName=ps_output  LeftPortType=input  RightPortType=output  PseudoPeriodic=off  Frequencies=[]  VectorFormat=inherit  Unit=rad/s  AffineConversion=off
  BallVxToSL : nesl_utility/PS-Simulink Converter  PhysicalDomain=network_engine_domain  SubClassName=ps_output  LeftPortType=input  RightPortType=output  PseudoPeriodic=off  Frequencies=[]  VectorFormat=inherit  Unit=m/s  AffineConversion=off
  BallVyToSL : nesl_utility/PS-Simulink Converter  PhysicalDomain=network_engine_domain  SubClassName=ps_output  LeftPortType=input  RightPortType=output  PseudoPeriodic=off  Frequencies=[]  VectorFormat=inherit  Unit=m/s  AffineConversion=off
  BallVzToSL : nesl_utility/PS-Simulink Converter  PhysicalDomain=network_engine_domain  SubClassName=ps_output  LeftPortType=input  RightPortType=output  PseudoPeriodic=off  Frequencies=[]  VectorFormat=inherit  Unit=m/s  AffineConversion=off
  GroundContactStatus : nesl_utility/PS-Simulink Converter  PhysicalDomain=network_engine_domain  SubClassName=ps_output  LeftPortType=input  RightPortType=output  PseudoPeriodic=off  Frequencies=[]  VectorFormat=inherit  Unit=1  AffineConversion=off
  TmpT : sm_lib/Frames and Transforms/Rigid Transform  RotationMethod=None  FollAlignAxisA=+X  BaseAlignAxisA=+Y  FollAlignAxisB=+Y  BaseAlignAxisB=+Z  RotationStandardAxis=+Z  RotationAngle=0  RotationAngleUnits=deg  RotationArbitraryAxis=[0 0 1]  RotationSequenceAxes=FollowerAxes  RotationSequence=XYX  RotationSequenceAngles=[0 0 0]  RotationSequenceAnglesUnits=deg  RotationMatrix=[1 0 0;0 1 0;0 0 1]  Quaternion=[1 0 0 0]  TranslationMethod=None  TranslationCartesianOffset=[0 0 0]  TranslationCartesianOffsetUnits=m  TranslationStandardAxis=+Z  TranslationStandardOffset=0  TranslationStandardOffsetUnits=m  TranslationROffset=0  TranslationROffsetUnits=m  TranslationThetaOffset=0  TranslationThetaOffsetUnits=deg  TranslationZOffset=0  TranslationZOffsetUnits=m
  Conn3 : PMIOPort  Side=Right
  Conn4 : PMIOPort  Port=2  Side=Left
  Conn5 : PMIOPort  Port=3  Side=Left
  output : Outport
  output1 : Outport  Port=2
  output2 : Outport  Port=3
  output3 : Outport  Port=4
  output4 : Outport  Port=5
  wires:
  BallPositionY/1 -> output2/1
  BallQuaternion/1 -> output4/1
  BallPositionZ/1 -> output3/1
  GroundContactStatus/1 -> output/1
  BallPositionX/1 -> output1/1
  BallVxToSL/1 -> BallRollResMux/1
  BallVyToSL/1 -> BallRollResMux/2
  BallVzToSL/1 -> BallRollResMux/3
  BallSpinToSL/1 -> BallRollResMux/4
  BallNormalToSL/1 -> BallRollResMux/5
  BallRollResMux/1 -> BallRollResFcn/1
  BallRollResFcn/1 -> BallRollResDemux/1
  BallRollResDemux/1 -> BallRollResForceToPS/1
  BallRollResDemux/2 -> BallRollResTorqueToPS/1
  connections:
  BallFreeJoint/RConn4 -- BallPositionY/LConn1
  BallFreeJoint/RConn6 -- BallPositionZ/LConn1
  BallSolid/RConn1 -- BallFreeJoint/RConn1 -- BallRollingLoad/RConn1
  BallGroundContact/RConn2 -- GroundContactStatus/LConn1
  BallFreeJoint/RConn8 -- BallQuaternion/LConn1
  BallFreeJoint/RConn2 -- BallPositionX/LConn1
  Conn3/RConn1 -- BallGroundContact/RConn1
  Conn4/RConn1 -- BallGroundContact/LConn1 -- BallSolid/LConn1
  Conn5/RConn1 -- BallFreeJoint/LConn1
  BallFreeJoint/RConn3 -- BallVxToSL/LConn1
  BallFreeJoint/RConn5 -- BallVyToSL/LConn1
  BallFreeJoint/RConn7 -- BallVzToSL/LConn1
  BallFreeJoint/RConn9 -- BallSpinToSL/LConn1
  BallGroundContact/RConn3 -- BallNormalToSL/LConn1
  BallRollResForceToPS/RConn1 -- BallRollingLoad/LConn1
  BallRollResTorqueToPS/RConn1 -- BallRollingLoad/LConn2

== system ball_balancing_omni3_multibody_lqi_rev1_r2024b/MultibodyPlant/Environment ==
  GroundFrame : sm_lib/Frames and Transforms/Rigid Transform  RotationMethod=None  FollAlignAxisA=+X  BaseAlignAxisA=+Y  FollAlignAxisB=+Y  BaseAlignAxisB=+Z  RotationStandardAxis=+Z  RotationAngle=0  RotationAngleUnits=deg  RotationArbitraryAxis=[0 0 1]  RotationSequenceAxes=FollowerAxes  RotationSequence=XYX  RotationSequenceAngles=[0 0 0]  RotationSequenceAnglesUnits=deg  RotationMatrix=[1 0 0;0 1 0;0 0 1]  Quaternion=[1 0 0 0]  TranslationMethod=None  TranslationCartesianOffset=[0 0 0]  TranslationCartesianOffsetUnits=m  TranslationStandardAxis=+Z  TranslationStandardOffset=0  TranslationStandardOffsetUnits=m  TranslationROffset=0  TranslationROffsetUnits=m  TranslationThetaOffset=0  TranslationThetaOffsetUnits=deg  TranslationZOffset=0  TranslationZOffsetUnits=m
  GroundPlane : sm_lib/Curves and Surfaces/Infinite Plane  GraphicType=Rectangle  GraphicPlaneWidth=2  GraphicPlaneWidthUnits=m  GraphicPlaneHeight=2  GraphicPlaneHeightUnits=m  GraphicVisPropType=SimpleVisualProperties  GraphicDiffuseColor=[0.5 0.5 0.5]  GraphicOpacity=1  GraphicSpecularColor=[0.5 0.5 0.5 1.0]  GraphicAmbientColor=[0.15 0.15 0.15 1.0]  GraphicEmissiveColor=[0.0 0.0 0.0 1.0]  GraphicShininess=75
  MechanismConfig : sm_lib/Utilities/Mechanism Configuration  UniformGravity=Constant  GravityVector=[0 0 -ballbotParams.gravity]  GravityVectorUnits=m/s^2  LinearizationDelta=0.001  JointModeTransitionNonlinearIterations=2
  SolverConfig : nesl_utility/Solver Configuration  PhysicalDomain=network_engine_domain  SubClassName=solver  LeftPortType=input  RightPortType=generic  Tones=[]  Harmonics=[]  SimulateNoise=off  Profile=off  UseLocalSampling=off  EnableSwitchedLinearOptims=on  FrequencyDomain=off  UseCCode=off  RelTol=0.001  AbsTol=0.001  MinStep=1e-09  ToWorkspace=off  RevertToSquareIcSolve=off  NumHomotopyIterations=100  PhasorMode=off  PhasorModeNumHarmonics=1  ConsistencySolver=NEWTON_XTOL_AFTER_FTOL  CanonicalOrdering=CANONICAL  OptimizeIntermediates=OPTIMIZED  IndexReductionMethod=DerivativeReplacement  DoDC=off  ResidualTolerance=1e-09  ConsistencyTolSource=GLOBAL  ConsistencyAbsTol=0.001  ConsistencyRelTol=0.001  ConsistencyTolFactor=0.001  UseLocalSolver=off  LocalSolverChoice=NE_BACKWARD_EULER_ADVANCER  ResolveIndetEquations=on  FunctionEvalNumThread=1  LocalSolverSampleTime=0.001  DoFixedCost=off  MaxNonlinIter=3  MaxModeIter=2  ComputeImpulses=off  ImpulseIterations=2  LinearAlgebra=auto  LinearAlgebraNumThread=0  EquationFormulation=NE_TIME_EF  DelaysMemoryBudget=1024  AutomaticFiltering=on  FilteringTimeConstant=0.001  PartitionStorageMethod=AS_NEEDED  PartitionMemoryBudget=1024  PartitionMethod=ROBUST  MultibodyUseLocalSolver=off  MultibodyLocalSolverChoice=ODE1  MultibodyLocalSolverSampleTime=0.001
  World : sm_lib/Frames and Transforms/World Frame
  port : PMIOPort  Side=Right
  Conn2 : PMIOPort  Port=2  Side=Left
  Conn3 : PMIOPort  Port=3  Side=Right
  Conn4 : PMIOPort  Port=4  Side=Right
  connections:
  GroundPlane/RConn1 -- Conn3/RConn1
  World/RConn1 -- Conn4/RConn1 -- MechanismConfig/RConn1
  Conn2/RConn1 -- GroundFrame/LConn1
  GroundFrame/RConn1 -- GroundPlane/LConn1
  SolverConfig/RConn1 -- port/RConn1
